simulink model "hdlcodercpu_eml"  (R2026a)
settings: Solver=FixedStepDiscrete  StopTime=20000
libraries: hdlsllib x1
Description:
  | 8-bit RISC Processor using MATLAB(R) Function Blocks
  | This model shows how to use Simulink(R) HDL Coder(TM) to check,
  | generate and verify HDL for an 8-bit CPU implemented using the
  | MATLAB Function Block.
settings Model: ExtModeAutoUpdateStatusClock=off  Creator=The MathWorks, Inc.  LastModifiedBy=The MathWorks, Inc.
settings SolverCC: InsertRTBMode=Auto
settings OptimizationCC: ConditionallyExecuteInputs=off  InitFltsAndDblsToZero=on  EfficientMapNaN2IntZero=off
settings DebuggingCC: AlgebraicLoopMsg=error  UnderspecifiedInitializationDetection=Classic  SingleTaskRateTransMsg=error
settings HardwareCC: ProdHWDeviceType=ASIC/FPGA->ASIC/FPGA  ProdEqTarget=off
settings GRTTargetCC: TargetFcnLib=ansi_tfl_tmw.mat  CombineOutputUpdateFcns=off  GRTInterface=on
settings ConfigComp: DVMaxProcessTime=600.0  DVAutomaticStubbing=off  DVParameterConfiguration=UseParameterConfigFile  DVParameters=on  DVModelCoverageObjectives=MCDC  DVMaxTestCaseSteps=500.0  DVTestSuiteOptimization=Auto  DVAbsoluteTolerance=1.0e-5  DVDefectChecker=off  DVDetectActiveLogic=on  DVMaxViolationSteps=20.0  DVSaveHarnessModel=on  DVModelReferenceHarness=on  DVHarnessSource=Signal Editor  DVSaveReport=on  DVActiveTab=0.0

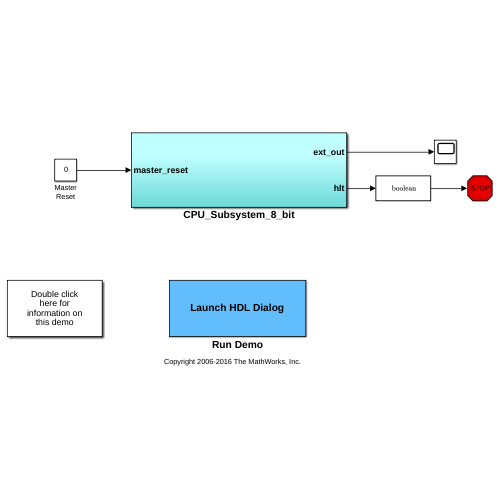
[thumbnail: Simulink's stored preview of the top-level diagram]
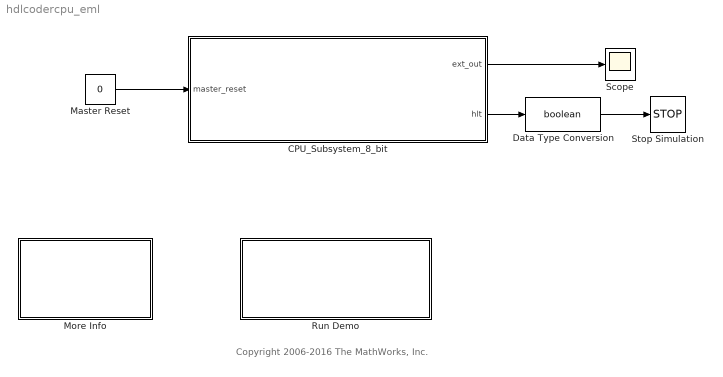
== system hdlcodercpu_eml ==
  note: Copyright 2006-2016 The MathWorks, Inc.
  CPU_Subsystem_8_bit : Subsystem
  Data Type Conversion : DataTypeConversion  OutDataTypeStr=boolean  SaturateOnIntegerOverflow=off  RndMeth=Floor
  Master Reset : Constant  Value=0  OutDataTypeStr=boolean  SampleTime=1
  More Info : Subsystem
      mask Display: disp('Double click\nhere for\ninformation on\nthis demo')
  Run Demo : Subsystem
      settings: OpenFcn=hdldialog(bdroot)
      mask Display: disp('Launch HDL Dialog')
  Scope : Scope
      settings: TimeSpan=100  ActiveDisplayYMinimum=0  ActiveDisplayYMaximum=7  DataLoggingMaxPoints=8500
  Stop Simulation : Stop
  wires:
  CPU_Subsystem_8_bit/1(ext_out) -> Scope/1
  CPU_Subsystem_8_bit/2(hlt) -> Data Type Conversion/1
  Data Type Conversion/1 -> Stop Simulation/1
  Master Reset/1 -> CPU_Subsystem_8_bit/1(master_reset)

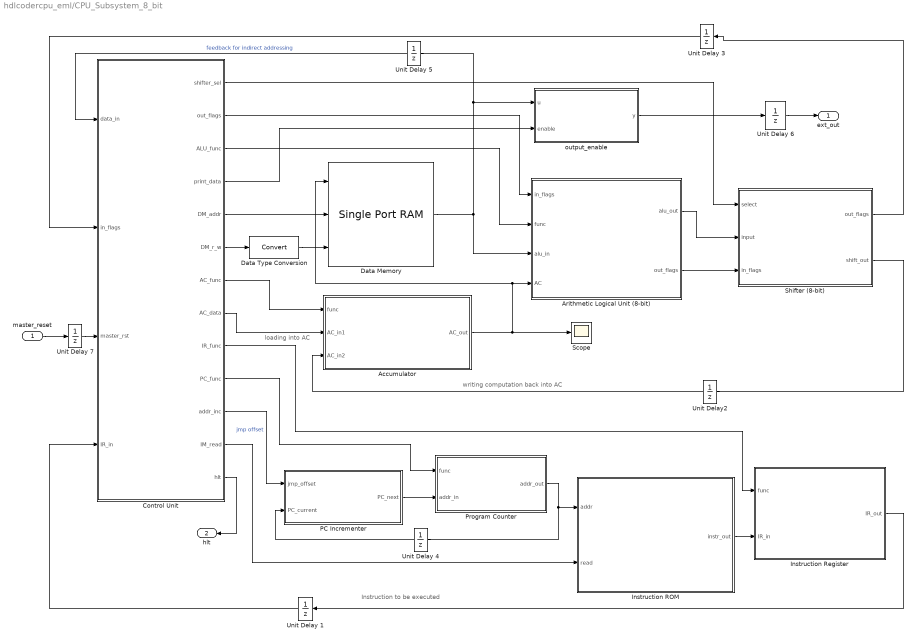
== system hdlcodercpu_eml/CPU_Subsystem_8_bit ==
  note: loading into AC
  note: writing computation back into AC
  note: Instruction to be executed
  master_reset : Inport
  Accumulator : MATLAB Function  TreatAsAtomicUnit=on
  Arithmetic Logical Unit (8-bit) : MATLAB Function  TreatAsAtomicUnit=on
  Control Unit : MATLAB Function  TreatAsAtomicUnit=on
  Data Memory : hdlsllib/HDL RAMs/Single Port RAM  ram_size=8  dout_type=New data
  Data Type Conversion : DataTypeConversion  SaturateOnIntegerOverflow=off  RndMeth=Floor
  Instruction ROM : MATLAB Function  TreatAsAtomicUnit=on
  Instruction Register : MATLAB Function  TreatAsAtomicUnit=on
  PC Incrementer : MATLAB Function  TreatAsAtomicUnit=on
  Program Counter : MATLAB Function  TreatAsAtomicUnit=on
  Scope : Scope
  Shifter (8-bit) : MATLAB Function  TreatAsAtomicUnit=on
  Unit Delay {1,3..7} (6 alike) : UnitDelay
  Unit Delay2 : UnitDelay
  output_enable : MATLAB Function  TreatAsAtomicUnit=on
  ext_out : Outport
  hlt : Outport  Port=2
  wires:
  Arithmetic Logical Unit (8-bit)/1(alu_out) -> Shifter (8-bit)/2(input)
  Arithmetic Logical Unit (8-bit)/2(out_flags) -> Shifter (8-bit)/3(in_flags)
  Accumulator/1(AC_out) -> Arithmetic Logical Unit (8-bit)/4(AC), Data Memory/1, Scope/1
  Data Memory/1 -> Arithmetic Logical Unit (8-bit)/3(alu_in), output_enable/1(u), Unit Delay 5/1
  Program Counter/1(addr_out) -> Instruction ROM/1(addr), Unit Delay 4/1
  PC Incrementer/1(PC_next) -> Program Counter/2(addr_in)
  Instruction ROM/1(instr_out) -> Instruction Register/2(IR_in)
  Control Unit/3(ALU_func) -> Arithmetic Logical Unit (8-bit)/2(func)
  Control Unit/1(shifter_sel) -> Shifter (8-bit)/1(select)
  Control Unit/2(out_flags) -> Arithmetic Logical Unit (8-bit)/1(in_flags)
  Control Unit/6(DM_r_w) -> Data Type Conversion/1
  Control Unit/7(AC_func) -> Accumulator/1(func)
  Control Unit/9(IR_func) -> Instruction Register/1(func)
  Control Unit/10(PC_func) -> Program Counter/1(func)
  Control Unit/11(addr_inc) -> PC Incrementer/1(jmp_offset)  "jmp offset"
  Control Unit/12(IM_read) -> Instruction ROM/2(read)
  Instruction Register/1(IR_out) -> Unit Delay 1/1
  Shifter (8-bit)/2(shift_out) -> Unit Delay2/1
  Unit Delay2/1 -> Accumulator/3(AC_in2)
  Unit Delay 4/1 -> PC Incrementer/2(PC_current)
  Control Unit/8(AC_data) -> Accumulator/2(AC_in1)
  master_reset/1 -> Unit Delay 7/1
  Control Unit/4(print_data) -> output_enable/2(enable)
  Control Unit/13(hlt) -> hlt/1
  Unit Delay 5/1 -> Control Unit/1(data_in)  "feedback for indirect addressing"
  output_enable/1(y) -> Unit Delay 6/1
  Data Type Conversion/1 -> Data Memory/3
  Control Unit/5(DM_addr) -> Data Memory/2
  Unit Delay 6/1 -> ext_out/1
  Unit Delay 7/1 -> Control Unit/3(master_rst)
  Unit Delay 3/1 -> Control Unit/2(in_flags)
  Unit Delay 1/1 -> Control Unit/4(IR_in)
  Shifter (8-bit)/1(out_flags) -> Unit Delay 3/1

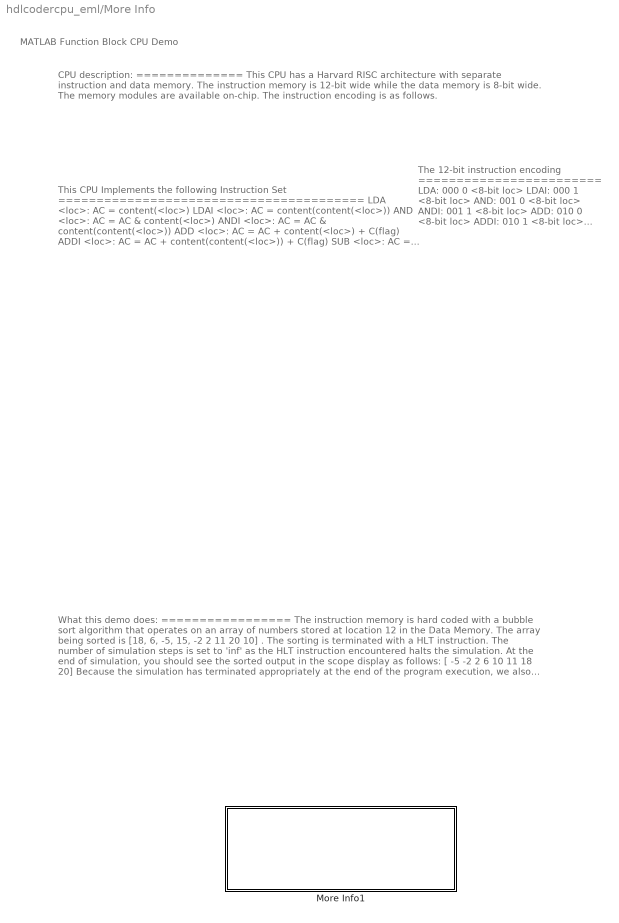
== system hdlcodercpu_eml/More Info ==
  note: MATLAB Function Block CPU Demo
  note: This CPU Implements the following Instruction Set
      | ========================================
      |
      | LDA <loc>: AC = content(<loc>)
      | LDAI <loc>: AC = content(content(<loc>))
      | AND <loc>: AC = AC & content(<loc>)
      | ANDI <loc>: AC = AC & content(content(<loc>))
      | ADD <loc>: AC = AC + content(<loc>) + C(flag)
      | ADDI <loc>: AC = AC + content(content(<loc>)) + C(flag)
      | SUB <loc>: AC = AC - content(<loc>) - C(flag)
      | SUBI <loc>: AC = AC - content(content(<loc>)) - C(flag)
      | JMP <loc>: Jump to <PC + <loc>>
      | LI <const>: AC = <const>
      | STA <loc>: content(<loc>) = AC
      | STAI <loc>: content(content(<loc>)) = AC
      | BRA_C <loc>: Jump to <PC + <loc>> if (C(flag) == 1)
      | BRA_N <loc>: Jump to <PC + <loc>> if (N(flag) == 1)
      | BRA_V <loc>: Jump to <PC + <loc>> if (V(flag) == 1)
      | BRA_Z <loc>: Jump to <PC + <loc>> if (Z(flag) == 1)
      | HLT: Halt (simulation)
      | CLA: AC = 0
      | CMA: Complement AC
      | CMC: Complement C(flag)
      | ASL: AC = AC << 1
      | ASR: AC = AC >> 1
      | PRINT: Display value from the memory-mapped location 255
      | CLC: C(flag) = 0
  note: The 12-bit instruction encoding
      | ========================
      |
      | LDA:     000 0 <8-bit loc>
      | LDAI:    000 1 <8-bit loc>
      | AND:     001 0 <8-bit loc>
      | ANDI:    001 1 <8-bit loc>
      | ADD:     010 0 <8-bit loc>
      | ADDI:    010 1 <8-bit loc>
      | SUB:     011 0 <8-bit loc>
      | SUBI:    011 1 <8-bit loc>
      | JMP:     1000 <8-bit loc>
      | LI:         1001 <8-bit const>
      | STA:     101 0 <8-bit loc>
      | STAI:    101 1 <8-bit loc>
      | BRA_C: 1100 <8-bit loc>
      | BRA_N: 1101 <8-bit loc>
      | BRA_C: 1110 <8-bit loc>
      | BRA_C: 1111 <8-bit loc>
      | HLT:     111 0 0100 0 000
      | CLA:      111 0 0100 1 000
      | CMA:     111 0 0101 0 000
      | CMC:     111 0 0101 1 000
      | ASL:      111 0 0110 0 000
      | ASR:      111 0 0110 1 000
      | PRINT:  111 0 0111 0 000
      | CLC:      111 0 0111 1 000
  note: CPU description:
      | ==============
      |
      | This CPU has a Harvard RISC architecture with separate instruction and data memory.
      | The instruction memory is 12-bit wide while the data memory is 8-bit wide.
      | The memory modules are available on-chip. The instruction encoding is as follows.
  note: What this demo does:
      | =================
      | The instruction memory is hard coded with a bubble sort algorithm that operates on an array
      | of numbers stored at location 12 in the Data Memory. The array being sorted is
      | [18, 6, -5, 15, -2 2 11 20 10] . The sorting is terminated with a HLT instruction.
      |
      | The number of simulation steps is set to 'inf' as the HLT instruction encountered halts the
      | simulation. At the end of simulation, you should see the sorted output in the scope display
      | as follows: [ -5 -2 2 6 10 11 18 20]
      |
      | Because the simulation has terminated appropriately at the end of the program execution,
      | we also get the number of time steps needed to execute the program.
  More Info1 : Subsystem
      mask Display: disp('Details of the Instruction memory\nthat contains a bubble sort algorithm')

== system hdlcodercpu_eml/Run Demo ==

== system hdlcodercpu_eml/More Info/More Info1 ==
  note: Bubble Sort
      | =========
      |
      | % Array Size
      |   LI 10     %  n = 10
      |   STA 0     %  n in loc 0
      |
      | % Array Pointer
      |   LI 12      %  loc 12 = starting location of a[]
      |   STA 1     %  loc 1 stores i which points to a[]
      |
      | % Array Entries begin in loc 12
      |   LI 18
      |   STA 12   % entry 1
      |   LI 6
      |   STA 13   % entry 2
      |   LI 19
      |   STA 14   % entry 3
      |   LI -5
      |   STA 15   % entry 4
      |   LI 15
      |   STA 16   % entry 5
      |   LI -2
      |   STA 17   % entry 6
      |   LI 2
      |   STA 18   % entry 7
      |   LI 11
      |   STA 19   % entry 8
      |   LI 20
      |   STA 20   % entry 9
      |   LI 10
      |   STA 21   % entry 10
      | L1:
      |   LI 1
      |   STA 2     %  loc 2 keeps track of count
      |   LI 1
      |   STA 3     %  loc 3 contains a predicate to flag the end of sorting
      | L2:
      | % accessing a[i-1]
      |   LI 1
      |   STA 4
      |   LDA 2
      |   CLC
      |   SUB 4    % i-1
      |   CLC
      |   ADD 1
      |   STA 5   % storing i-1 in loc 5
      |   LDAI 5   % a[i-1]
      |   STA 6    % temporarily storing a[i-1] in loc 6
      | % accessing a[i]
      |   LDA 2
      |   CLC
      |   ADD 1
      |   STA 7   % storing i in loc 7
      |   LDAI 7   % a[i]
      |   CLC
      |   SUB 6  % a[i] - a[i-1]
      |   BRA_N L5
      |   % a[i] >= a[i-1]
      |   JMP L6
  note: Bubble Sort     (continued)
      | =========
      |  L5:
      |    % a[i-1] > a[i]
      |  %  reset the flag indicating further sorting passes are reqd
      |    LI 0
      |    STA 3
      |  % Swapping a[i] and a[i-1]
      |    LDAI 7   % a[i]
      |    STAI 5   % a[i-1] = a[i]
      |    LDA 6   % temp
      |    STAI 7   % a[i] = temp
      |  L6:
      |    LI 1
      |    CLC
      |    ADD 2
      |    STA 2     %  count = count + 1
      |    LDA 0
      |    CLC
      |    SUB 2    %  AC = n - count
      |    BRA_Z L3    %  Break out of loop if count == n
      |    JMP L2
      |  L3:
      |    LI 1
      |    STA 4
      |    LDA 3
      |    CLC
      |    SUB 4
      |    BRA_Z L4    %  if flag == 1 indicating sorting over, break out
      |    JMP L1
      |  L4:
      |    LI 0
      |    STA 2     %  loc 2 keeps track of count
      |  % Printing the array
      |  L7:
      |    LDAI 1   % load a[i]
      |    STA 255
      |    PRINT     %  printing a[i]
      |    LI 1
      |    CLC
      |    ADD 1
      |    STA 1     %  i = i + 1
      |    LI 1
      |    CLC
      |    ADD 2
      |    STA 2     %  count = count + 1
      |    LDA 0
      |    CLC
      |    SUB 2    %  AC = n - count
      |    BRA_Z L8    %  Break out of loop if count == n
      |    JMP L7    %  Looping around
      |  L8:
      |    HLT
  note: The following program is hardcoded in
      | hdlcodercpu_eml/CPU Subsystem (8-bit)/Instruction ROM

== matlab function hdlcodercpu_eml/CPU_Subsystem_8_bit/PC Incrementer ==
  settings: updateMethod=DISCRETE  sampleTime=1
  settings: fimath=|
      | fimath(...
      | 'RoundMode', 'floor',...
      | 'OverflowMode', 'wrap',...
      | 'ProductMode', 'FullPrecision', 'ProductWordLength', 32,...
      | 'SumMode', 'FullPrecision', 'SumWordLength', 32,...
      | 'CastBeforeSum', true)
  data: jmp_offset input fixdt(1,8,0); PC_current input fixdt(0,8,0); PC_next output
function PC_next  = PC_Inc(jmp_offset, PC_current)
% PC incrementer increments the PC with jmp_offset

% HDL specific fimath
hdl_fm = fimath(...
'RoundMode', 'floor',...
'OverflowMode', 'wrap',...
'ProductMode', 'FullPrecision', 'ProductWordLength', 32,...
'SumMode', 'FullPrecision', 'SumWordLength', 32,...
'CastBeforeSum', true);

PC_next = fi(jmp_offset + PC_current, 0, 8, 0, hdl_fm);

== matlab function hdlcodercpu_eml/CPU_Subsystem_8_bit/output_enable ==
  data: u input fixdt(1,8,0); y output; enable input
function y = output_enable(u, enable)
% to the pin-out

% HDL specific fimath
hdl_fm = fimath(...
'RoundMode', 'floor',...
'OverflowMode', 'wrap',...
'ProductMode', 'FullPrecision', 'ProductWordLength', 32,...
'SumMode', 'FullPrecision', 'SumWordLength', 32,...
'CastBeforeSum', true);

y = fi(0, 1, 8, 0, hdl_fm);

if(enable)
    y = fi(u, 1, 8, 0, hdl_fm);
end

== matlab function hdlcodercpu_eml/CPU_Subsystem_8_bit/Control Unit ==
  settings: updateMethod=DISCRETE  sampleTime=1
  settings: fimath=|
      | fimath(...
      | 'RoundMode', 'floor',...
      | 'OverflowMode', 'wrap',...
      | 'ProductMode', 'FullPrecision', 'ProductWordLength', 32,...
      | 'SumMode', 'FullPrecision', 'SumWordLength', 32,...
      | 'CastBeforeSum', true)
  data: data_in input fixdt(1,8,0); in_flags input fixdt(0,4,0); master_rst input; shifter_sel output; out_flags output; ALU_func output; print_data output; IR_in input fixdt(0,12,0); DM_addr output; DM_r_w output; AC_func output; AC_data output; IR_func output; PC_func output; addr_inc output; IM_read output; hlt output
function [shifter_sel, out_flags, ALU_func, ...
    print_data, DM_addr, DM_r_w, AC_func, AC_data, IR_func, ...
    PC_func, addr_inc, IM_read, hlt] = Controller(data_in, in_flags, master_rst, IR_in)
% CPU Controller
%
% The CPU Instruction Set:
% ------------------------
% 
% LDA <loc>: AC = content(<loc>)
% LDAI <loc>: AC = content(content(<loc>))
% AND <loc>: AC = AC & content(<loc>)
% ANDI <loc>: AC = AC & content(content(<loc>))
% ADD <loc>: AC = AC + content(<loc>) + C(flag) 
% ADDI <loc>: AC = AC + content(content(<loc>)) + C(flag)
% SUB <loc>: AC = AC - content(<loc>) - C(flag) 
% SUBI <loc>: AC = AC - content(content(<loc>)) - C(flag)
% JMP <loc>: Jump to <PC + <loc>>
% LI <const>: AC = <const>
% STA <loc>: content(<loc>) = AC
% STAI <loc>: content(content(<loc>)) = AC
% BRA_C <loc>: Jump to <PC + <loc>> if (C(flag) == 1)
% BRA_N <loc>: Jump to <PC + <loc>> if (N(flag) == 1)
% BRA_V <loc>: Jump to <PC + <loc>> if (V(flag) == 1)
% BRA_Z <loc>: Jump to <PC + <loc>> if (Z(flag) == 1)
% NOP: Do nothing
% CLA: AC = 0
% CMA: Complement AC
% CMC: Complement C(flag)
% ASL: AC = AC << 1
% ASR: AC = AC >> 1
% PRINT: Display value from the memory-mapped location 255
% CLC: C(flag) = 0
%
% 12-bit Instruction Encoding:
% ---------------------------
%
% 	LDA:   000 0 <8-bit loc>
% 	LDAI:  000 1 <8-bit loc>
% 	AND:   001 0 <8-bit loc>
% 	ANDI:  001 1 <8-bit loc>
% 	ADD:   010 0 <8-bit loc>
% 	ADDI:  010 1 <8-bit loc>
% 	SUB:   011 0 <8-bit loc>
% 	SUBI:  011 1 <8-bit loc>
% 	JMP:   1000 <8-bit loc>
% 	LI:    1001 <8-bit const>
% 	STA:   101 0 <8-bit loc>
% 	STAI:  101 1 <8-bit loc>
% 	BRA_C: 1100 <8-bit loc>
% 	BRA_N: 1101 <8-bit loc>
% 	BRA_C: 1110 <8-bit loc>
% 	BRA_C: 1111 <8-bit loc>
% 	HLT:   111 0 0100 0 000 
% 	CLA:   111 0 0100 1 000
% 	CMA:   111 0 0101 0 000
% 	CMC:   111 0 0101 1 000
% 	ASL:   111 0 0110 0 000
% 	ASR:   111 0 0110 1 000
% 	PRINT: 111 0 0111 0 000
% 	CLC:   111 0 0111 1 000  

% HDL specific fimath
hdl_fm = fimath(...
'RoundMode', 'floor',...
'OverflowMode', 'wrap',...
'ProductMode', 'FullPrecision', 'ProductWordLength', 32,...
'SumMode', 'FullPrecision', 'SumWordLength', 32,...
'CastBeforeSum', true);


persistent CPU_state;
if(isempty(CPU_state))
    CPU_state = uint8(0);
end

persistent previous_CPU_state;
if(isempty(previous_CPU_state))
    previous_CPU_state = uint8(0);
end

if(master_rst)
    CPU_state = uint8(0);
end

shifter_sel = fi(0, 0, 2, 0, hdl_fm);
ALU_func = fi(0, 0, 3, 0, hdl_fm);
out_flags = in_flags;
AC_func = fi(4, 0, 3, 0, hdl_fm);  % NOP
AC_data = fi(0, 1, 8, 0, hdl_fm);
IR_func = fi(3, 0, 2, 0, hdl_fm);  % NOP
PC_func = fi(3, 0, 2, 0, hdl_fm);  % NOP
IM_read = fi(0, 0, 1, 0, hdl_fm);
DM_addr = fi(0, 0, 8, 0, hdl_fm); % uint8(0)
DM_r_w = fi(0, 0, 1, 0, hdl_fm);
addr_inc = fi(0, 1, 8, 0, hdl_fm);
print_data = false;
hlt = uint8(0);

% Instruction: <12..1>
% major_opcode: <12..10>
% indirect_addressing: <9>
% minor_opcode: <9..4>
% address bits: <8..1>

persistent major_opcode; 
persistent minor_opcode; 
persistent address_data;
persistent indirect_address;

if(isempty(major_opcode))
    major_opcode = fi(0, 0, 8, 0, hdl_fm);
    minor_opcode = fi(0, 0, 8, 0, hdl_fm);
    address_data = fi(0, 0, 8, 0, hdl_fm);
    indirect_address = fi(0, 0, 8, 0, hdl_fm);
end

switch(CPU_state)
    %%%%%%%%%%%%%%%%%%%%%%%%%%%%%%%%%%%%%%
    %  RESETTING OUTPUTS
    %%%%%%%%%%%%%%%%%%%%%%%%%%%%%%%%%%%%%%
    case 0
        PC_func = fi(0, 0, 2, 0, hdl_fm);   
        AC_func = fi(0, 0, 3, 0, hdl_fm);   
        IR_func = fi(0, 0, 2, 0, hdl_fm);   
        previous_CPU_state = CPU_state;
        CPU_state = uint8(1);
        
    %%%%%%%%%%%%%%%%%%%%%%%%%%%%%%%%%%%%%%
    %  FETCH
    %%%%%%%%%%%%%%%%%%%%%%%%%%%%%%%%%%%%%%
    case 1  
        % Read from IM
        IM_read = fi(1, 0, 1, 0, hdl_fm);  
        % Increment PC
        PC_func = fi(2, 0, 2, 0, hdl_fm);  
        % store into IR
        IR_func = fi(1, 0, 2, 0, hdl_fm);  
        
        CPU_state = uint8(2);
        
    case 2 
        % Read from IR
        IR_func = fi(2, 0, 2, 0, hdl_fm);  
        % Accommodating for the 'unit delay' from IR_out to IR_in
        
        CPU_state = uint8(3);  
        
    case 3
        % IR_in <12..10>
        major_opcode = fi(bitsrl(IR_in, 9), 0, 8, 0, hdl_fm);
        mask = fi(63, 0, 12, 0, hdl_fm);
        % IR_in <9..4>
        minor_opcode = fi(bitand(bitsrl(IR_in, 3), mask), 0, 8, 0, hdl_fm);
        mask = fi(255, 0, 12, 0, hdl_fm);
        % IR_in <8..1>
        address_data = fi(bitand(IR_in, mask), 0, 8, 0, hdl_fm);
        
        % Go to the decode stage
        CPU_state = uint8(4);  
        
    %%%%%%%%%%%%%%%%%%%%%%%%%%%%%%%%%%%%%%
    %  DECODE AND EXECUTE
    %%%%%%%%%%%%%%%%%%%%%%%%%%%%%%%%%%%%%%
    case 4  
        previous_CPU_state = CPU_state;
        switch(uint8(major_opcode))
            case 0  
                % LDA
                % minor_opcode contains the address (assuming direct addressing)
                DM_addr = address_data; 
                % Read the data memory
                DM_r_w = fi(0, 0, 1, 0, hdl_fm); 
                % Simply pass the value read from memory
                CPU_state = uint8(13);
                
            case 1  
                % AND           
                DM_addr = address_data;
                % Reading the data memory for address or data
                DM_r_w = fi(0, 0, 1, 0, hdl_fm);
                
                CPU_state = uint8(15);
                
            case 2  
                % ADD
                DM_addr = address_data;
                % Reading the data memory for address or data
                DM_r_w = fi(0, 0, 1, 0, hdl_fm);
                
                CPU_state = uint8(17);
                
            case 3  
                % SUB
                DM_addr = address_data;
                % Reading the data memory for address or data
                DM_r_w = fi(0, 0, 1, 0, hdl_fm);
                
                CPU_state = uint8(19);

            case 4  
                minor_opcode_bit6 = bitget(minor_opcode, 6);
                switch(uint8(minor_opcode_bit6))
                    case 0 
                        % JMP
                        temp_address_data = fi(address_data, 1, 7, 0, hdl_fm);
                        addr_inc = fi(temp_address_data-1, 1, 8, 0, hdl_fm);
                        PC_func = fi(1, 0, 2, 0, hdl_fm); 
                        
                    case 1
                        % LI
                        AC_data = fi(address_data, 1, 8, 0, hdl_fm);
                        AC_func = fi(1, 0, 3, 0, hdl_fm);
                end
                % Go back to the fetch stage again
                CPU_state = uint8(1);  
                
            case 5  
                % STA
                % minor_opcode contains the address (assuming direct addressing)
                DM_addr = address_data; 
                indirect_bit = bitget(minor_opcode, 6);
                if(logical(indirect_bit))
                    % indirect addressing
                    % Read the address from the data memory
                    DM_r_w = fi(0, 0, 1, 0, hdl_fm); 
                    CPU_state = uint8(21);
                else
                    % Write into the data memory
                    DM_r_w = fi(1, 0, 1, 0, hdl_fm);
                    % Go back to the fetch stage again
                    CPU_state = uint8(25);  % going to 'otherwise'
                end
                
            case 6
                minor_opcode_bit6 = bitget(minor_opcode, 6);
                switch(uint8(minor_opcode_bit6))
                    % special branches:
                    case 0 
                        % BRA_C
                        c = bitget(in_flags, 4);
                        if(logical(c))
                            temp_address_data = fi(address_data, 1, 7, 0, hdl_fm);
                            addr_inc = fi(temp_address_data-1, 1, 8, 0, hdl_fm);
                            PC_func = fi(1, 0, 2, 0, hdl_fm);
                        end
                        
                    case 1
                        % BRA_N
                        n = bitget(in_flags, 3);
                        if(logical(n))
                            temp_address_data = fi(address_data, 1, 7, 0, hdl_fm);
                            addr_inc = fi(temp_address_data-1, 1, 8, 0, hdl_fm);
                            PC_func = fi(1, 0, 2, 0, hdl_fm);
                        end
                end
                % Go back to the fetch stage again
                CPU_state = uint8(15);
                
            case 7  
                 % by default, go back to the fetch stage again
                CPU_state = uint8(1);
                minor_opcode_bit4 = bitget(minor_opcode, 4);
                if(logical(minor_opcode_bit4) == 0)
                    % Further cases of special branches:
                    minor_opcode_bit6 = bitget(minor_opcode, 6);
                    switch(uint8(minor_opcode_bit6))
                        case 0 
                            % BRA_V
                            v = bitget(in_flags, 2);
                            if(logical(v))
                                temp_address_data = fi(address_data, 1, 7, 0, hdl_fm);
                                addr_inc = fi(temp_address_data-1, 1, 8, 0, hdl_fm);
                                PC_func = fi(1, 0, 2, 0, hdl_fm);
                            end
                         
                        case 1 
                            % BRA_Z
                            z = bitget(in_flags, 1);
                            if(logical(z))
                                temp_address_data = fi(address_data, 1, 7, 0, hdl_fm);
                                addr_inc = fi(temp_address_data-1, 1, 8, 0, hdl_fm);
                                PC_func = fi(1, 0, 2, 0, hdl_fm);
                            end
                    end
                end
                % Instructions having no operands
                switch(uint8(minor_opcode))
                    case 8
                        % HLT
                        % Stop the simulation
                        hlt = uint8(1);
                        CPU_state = uint8(22);
                    case 9 
                        % CLA
                        AC_func = fi(0, 0, 3, 0, hdl_fm);
                        
                    case 10 
                        % CMA
                        ALU_func = fi(4, 0, 3, 0, hdl_fm); 
                        shifter_sel = fi(3, 0, 2, 0, hdl_fm);
                        CPU_state = uint8(6);
                        
                    case 11 
                        % CMC
                        ALU_func = fi(5, 0, 3, 0, hdl_fm); 
                        shifter_sel = fi(3, 0, 2, 0, hdl_fm);
                        
                    case 12 
                        % ASL
                        shifter_sel = fi(1, 0, 2, 0, hdl_fm);
                        CPU_state = uint8(6);
                        
                    case 13 
                        % ASR
                        shifter_sel = fi(2, 0, 2, 0, hdl_fm);
                        CPU_state = uint8(6);
                        
                    case 14 
                        % PRINT   
                        DM_addr = fi(255, 0, 8, 0, hdl_fm);
                        % Read the data memory
                        DM_r_w = fi(0, 0, 1, 0, hdl_fm);
                        
                        CPU_state = uint8(12);

                    case 15 
                        % CLC
                        ALU_func = fi(7, 0, 3, 0, hdl_fm); 
                        shifter_sel = fi(3, 0, 2, 0, hdl_fm);
                        
                    otherwise
                        % by default, go back to the fetch stage again
                        CPU_state = uint8(1);
  
                % Minor Opcode cases end here        
                end
        % Major Opcode cases end here
        end
    
    % introducing delay
    case 6
        % accounting for the delay from shift_out to AC_in2
        AC_func = fi(2, 0, 3, 0, hdl_fm);
        previous_CPU_state = CPU_state;
        % Go back to the fetch stage again
        CPU_state = uint8(1);  
        
    % Operations with indirect addressing
    case 7
        % LDA Indirect
        % data_in is the address read from the data memory
        DM_addr = indirect_address; 
        % Read the data memory
        DM_r_w = fi(0, 0, 1, 0, hdl_fm); 
        
        previous_CPU_state = CPU_state;
        CPU_state = uint8(13);
        
    case 8
        % AND Indirect
        % data_in is the address read from the data memory
        DM_addr = indirect_address;
        % Read the data memory
        DM_r_w = fi(0, 0, 1, 0, hdl_fm);

        previous_CPU_state = CPU_state;
        CPU_state = uint8(15);
    
    case 9
        % ADD Indirect
        % data_in is the address read from the data memory
        DM_addr = indirect_address;
        % Read the data memory
        DM_r_w = fi(0, 0, 1, 0, hdl_fm);
        
        previous_CPU_state = CPU_state;
        CPU_state = uint8(17);
        
    case 10
        % SUB Indirect
        % data_in is the address read from the data memory
        DM_addr = indirect_address;
        % Read the data memory
        DM_r_w = fi(0, 0, 1, 0, hdl_fm);
        
        previous_CPU_state = CPU_state;
        CPU_state = uint8(19);
        
    case 11
        % STA Indirect
        % data_in is the address read from the data memory
        DM_addr = fi(data_in, 0, 8, 0, hdl_fm);
        % Write the data memory
        DM_r_w = fi(1, 0, 1, 0, hdl_fm);
        previous_CPU_state = CPU_state;
        CPU_state = uint8(1);
        
    case 12
        % PRINT
        print_data = true;
        previous_CPU_state = CPU_state;
        CPU_state = uint8(1);
        
    case 13
        % LDA (contd.)
        % Simply pass the value read from memory
        ALU_func = fi(6, 0, 3, 0, hdl_fm);
        shifter_sel = fi(3, 0, 2, 0, hdl_fm);

        if(previous_CPU_state == uint8(4))
            previous_CPU_state = CPU_state;
            CPU_state = uint8(14);
        else
            previous_CPU_state = CPU_state;
            CPU_state = uint8(6);
        end
        
    case 14
        indirect_bit = bitget(minor_opcode, 6);
        % accounting for the delay from shift_out to AC_in2
        AC_func = fi(2, 0, 3, 0, hdl_fm);
        
        previous_CPU_state = CPU_state;
        if(logical(indirect_bit))
            % indirect addressing
            indirect_address = fi(data_in, 0, 8, 0, hdl_fm);
            CPU_state = uint8(7);
        else
            CPU_state = uint8(25);
        end

    case 15

        % AND (contd.)
        ALU_func = fi(1, 0, 3, 0, hdl_fm);
        shifter_sel = fi(3, 0, 2, 0, hdl_fm);

        if(previous_CPU_state == uint8(4))
            previous_CPU_state = CPU_state;
            CPU_state = uint8(16);
        else
            previous_CPU_state = CPU_state;
            CPU_state = uint8(6);
        end

    case 16
        indirect_bit = bitget(minor_opcode, 6);
        % accounting for the delay from shift_out to AC_in2
        AC_func = fi(2, 0, 3, 0, hdl_fm);
        
        previous_CPU_state = CPU_state;
        if(logical(indirect_bit))
            % indirect addressing
            indirect_address = fi(data_in, 0, 8, 0, hdl_fm);
            CPU_state = uint8(8);
        else
            CPU_state = uint8(25);
        end
        
    case 17
        % ADD (contd.)
        ALU_func = fi(2, 0, 3, 0, hdl_fm);
        shifter_sel = fi(3, 0, 2, 0, hdl_fm);

        if(previous_CPU_state == uint8(4))
            previous_CPU_state = CPU_state;
            CPU_state = uint8(18);
        else
            previous_CPU_state = CPU_state;
            CPU_state = uint8(6);
        end

    case 18
        indirect_bit = bitget(minor_opcode, 6);
        % accounting for the delay from shift_out to AC_in2
        AC_func = fi(2, 0, 3, 0, hdl_fm);
        
        previous_CPU_state = CPU_state;
        if(logical(indirect_bit))
            % indirect addressing
            indirect_address = fi(data_in, 0, 8, 0, hdl_fm);
            CPU_state = uint8(9);
        else
            CPU_state = uint8(25);
        end
        
    case 19
        % SUB (contd.)
        ALU_func = fi(3, 0, 3, 0, hdl_fm);
        shifter_sel = fi(3, 0, 2, 0, hdl_fm);

        if(previous_CPU_state == uint8(4))
            previous_CPU_state = CPU_state;
            CPU_state = uint8(20);
        else
            previous_CPU_state = CPU_state;
            CPU_state = uint8(6);
        end

    case 20
        indirect_bit = bitget(minor_opcode, 6);
        % accounting for the delay from shift_out to AC_in2
        AC_func = fi(2, 0, 3, 0, hdl_fm);
        
        previous_CPU_state = CPU_state;
        if(logical(indirect_bit))
            % indirect addressing
            indirect_address = fi(data_in, 0, 8, 0, hdl_fm);
            CPU_state = uint8(10);
        else

            CPU_state = uint8(25);
        end
        
    case 21
        % STA indirect
        CPU_state = uint8(11);
        
    case 22
        % lock state
        hlt = uint8(1);
        CPU_state = uint8(22);

    otherwise
        previous_CPU_state = CPU_state;
        % by default, go back to the fetch stage again
        CPU_state = uint8(1);
                
% switch(CPU_state) end here
end

== matlab function hdlcodercpu_eml/CPU_Subsystem_8_bit/Accumulator ==
  settings: updateMethod=DISCRETE  sampleTime=1
  settings: fimath=|
      | fimath(...
      | 'RoundMode', 'floor',...
      | 'OverflowMode', 'wrap',...
      | 'ProductMode', 'FullPrecision', 'ProductWordLength', 32,...
      | 'SumMode', 'FullPrecision', 'SumWordLength', 32,...
      | 'CastBeforeSum', true)
  data: func input; AC_out output fixdt(1,8,0); AC_in1 input fixdt(1,8,0); AC_in2 input fixdt(1,8,0)

%% Accumulator with the following func:
% func == 0 => reset
% func == 1 => store into AC from port 1
% func == 2 => store into AC from port 2
% func == 3 => read from AC;
% otherwise, preserve old value and return 0
function AC_out = Accumulator(func, AC_in1, AC_in2)

% HDL specific fimath
hdl_fm = fimath(...
'RoundMode', 'floor',...
'OverflowMode', 'wrap',...
'ProductMode', 'FullPrecision', 'ProductWordLength', 32,...
'SumMode', 'FullPrecision', 'SumWordLength', 32,...
'CastBeforeSum', true);


persistent AC_value;
if(isempty(AC_value))
    AC_value = fi(0, 1, 8, 0, hdl_fm);
end

AC_out = fi(AC_value, 1, 8, 0, hdl_fm);
        
switch(uint8(func)) 
    case 0
        % reset
        AC_value = fi(0, 1, 8, 0, hdl_fm); 
    case 1 
        % store into AC
        AC_value = AC_in1;
    case 2
        % store into AC
        AC_value = AC_in2;    
    case 3
        % read the AC value
        AC_out = AC_value;
end

== matlab function hdlcodercpu_eml/CPU_Subsystem_8_bit/Arithmetic Logical Unit (8-bit) ==
  settings: updateMethod=DISCRETE  sampleTime=1
  settings: fimath=|
      | fimath(...
      | 'RoundMode', 'floor',...
      | 'OverflowMode', 'wrap',...
      | 'ProductMode', 'FullPrecision', 'ProductWordLength', 32,...
      | 'SumMode', 'FullPrecision', 'SumWordLength', 32,...
      | 'CastBeforeSum', true)
  data: in_flags input fixdt(0,4,0); func input fixdt(0,3,0); alu_in input fixdt(1,8,0); AC input fixdt(1,8,0); alu_out output fixdt(1,8,0); out_flags output
function [alu_out, out_flags] = ALU(in_flags, func, alu_in, AC)
% This 8-bit ALU supports the following operations:
% AND (Logical AND), ADD, SUB, CMA (Complement AC), CMC (Complement Carry) and CLC (Clear Carry)
% and appropriately sets a 4-bit flag register, which has the following format:
% [C N V Z]

% HDL specific fimath
hdl_fm = fimath(...
'RoundMode', 'floor',...
'OverflowMode', 'wrap',...
'ProductMode', 'FullPrecision', 'ProductWordLength', 32,...
'SumMode', 'FullPrecision', 'SumWordLength', 32,...
'CastBeforeSum', true);

% Get the carry in
carry = bitget(in_flags, 4); 

% Get the overflow in
overflow = bitget(in_flags, 2);

% Simply pass the AC, when there is no designated func
alu_out = fi(AC, 1, 8, 0, hdl_fm);

% 3-bit encoding of ALU ops, which can potentially support upto 8 operations
% Most of the encodings are unused to comply to Parwan supported ops
switch(uint8(func))
    case 0 % NOP
        % simply pass the AC
    case 1 % AND
        % Bitwise AND
        alu_out = bitand(alu_in, AC);
    case 2 % ADD
        % Add with carry and overflow appropriately set
        [alu_out, carry, overflow] = sum_w_carry(AC, alu_in, carry);
    case 3 % SUB
        % Subtract with borrow (set to carry) and overflow appropriately set
        [alu_out, carry, overflow] = sub_w_borrow(AC, alu_in, carry);
    case 4 % CMA
        % Complement AC
        alu_out = fi(bitcmp(AC), 1, 8, 0, hdl_fm);
    case 5 % CMC
        % Complement Carry
        carry = bitcmp(carry);
    case 6 % Get alu_in out
        % Pass the input
        alu_out = fi(alu_in, 1, 8, 0, hdl_fm);
    case 7 % CLC
        % Clear Carry
        carry = fi(0, 0, 1, 0, hdl_fm); 
end

% Negativity  (N)
sign_bit = getmsb(alu_out); 

% Is Zero? (Z)
is_zero = uint8(~all(alu_out));
zero_ufix1 = fi(is_zero, 0, 1, 0, hdl_fm);

% Set the output flag register [C N V Z]
out_flags = bitconcat(bitconcat(bitconcat(carry, sign_bit), overflow), zero_ufix1);

%%%%%%%%%%%%%%%%%%%%%%%%%%%%%%%%%%%%%%%%%%%%%%%%%%%%%%%%%%%%%%%%


%% Full Subtracter with flag register appropriately set 
% diff = u1 - u2 - b_in = u1 + bitcmp(u2) + bitcmp(b_in)
% appropriately set the borrow and the overflow
function [diff, carry, overflow] = sub_w_borrow(u1, u2, b_in)

[diff, carry, overflow] = sum_w_carry(u1, bitcmp(u2), bitcmp(b_in));
%%%%%%%%%%%%%%%%%%%%%%%%%%%%%%%%%%%%%%%%%%%%%%%%%%%%%%%%%%%%%%%%


%% Full Adder with flag register appropriately set
% sum = u1 + u2 + c_in
% appropriately set the carry and the overflow
function [sum, carry, overflow] = sum_w_carry(u1, u2, c_in)

hdl_fm = fimath(...
'RoundMode', 'floor',...
'OverflowMode', 'wrap',...
'ProductMode', 'FullPrecision', 'ProductWordLength', 32,...
'SumMode', 'FullPrecision', 'SumWordLength', 32,...
'CastBeforeSum', true);

% zero-extend u1 by 1 bit for carry detection
temp_u1 = fi(bitconcat(fi(0, 0, 1, 0, hdl_fm), u1), 1, 9, 0, hdl_fm);

% zero-extend u2 by 1 bit for carry detection
temp_u2 = fi(bitconcat(fi(0, 0, 1, 0, hdl_fm), u2), 1, 9, 0, hdl_fm);

% Sum is stored in 9 bits with the msb indicating carry
temp_sum = fi(temp_u1 + temp_u2 + c_in, 1, 9, 0, hdl_fm);

% Carry  (C)
carry = getmsb(temp_sum);

% Stored back in the designated register
sum = fi(temp_sum, 1, 8, 0, hdl_fm);

% Sign bit
sign_bit = getmsb(sum); 

% if the inputs have the same sign and the output generated has a different sign, 
% overflow is generated!
overflow_int = uint8((getmsb(u1) == getmsb(u2)) ...
                     && (sign_bit ~= bitget(u1,8)));
                 
% Overflow (V)
overflow = fi(overflow_int, 0, 1, 0, hdl_fm);

%%%%%%%%%%%%%%%%%%%%%%%%%%%%%%%%%%%%%%%%%%%%%%%%%%%%%%%%%%%%%%%%

== matlab function hdlcodercpu_eml/CPU_Subsystem_8_bit/Instruction ROM ==
  settings: updateMethod=DISCRETE  sampleTime=1
  settings: fimath=|
      | fimath(...
      | 'RoundMode', 'floor',...
      | 'OverflowMode', 'wrap',...
      | 'ProductMode', 'FullPrecision', 'ProductWordLength', 32,...
      | 'SumMode', 'FullPrecision', 'SumWordLength', 32,...
      | 'CastBeforeSum', true)
  data: addr input uint8; read input fixdt(0,1,0); instr_out output
function instr_out = Instr_Memory(addr, read)
%% Instruction Memory

% read == 1 => read from IM

% HDL specific fimath
hdl_fm = fimath(...
'RoundMode', 'floor',...
'OverflowMode', 'wrap',...
'ProductMode', 'FullPrecision', 'ProductWordLength', 32,...
'SumMode', 'FullPrecision', 'SumWordLength', 32,...
'CastBeforeSum', true);


persistent data;
if(isempty(data))
    data = fi(zeros(1, 256), 0, 12, 0, hdl_fm);
end

% ASSEMBLED CODE from sort1.in
data(1) = fi(2314, 0, 12, 0, hdl_fm);    % LI 10
data(2) = fi(2560, 0, 12, 0, hdl_fm);    % STA 0
data(3) = fi(2316, 0, 12, 0, hdl_fm);    % LI 12
data(4) = fi(2561, 0, 12, 0, hdl_fm);    % STA 1
data(5) = fi(2322, 0, 12, 0, hdl_fm);    % LI 18
data(6) = fi(2572, 0, 12, 0, hdl_fm);    % STA 12
data(7) = fi(2310, 0, 12, 0, hdl_fm);    % LI 6
data(8) = fi(2573, 0, 12, 0, hdl_fm);    % STA 13
data(9) = fi(2323, 0, 12, 0, hdl_fm);    % LI 19
data(10) = fi(2574, 0, 12, 0, hdl_fm);    % STA 14
data(11) = fi(2555, 0, 12, 0, hdl_fm);    % LI 251
data(12) = fi(2575, 0, 12, 0, hdl_fm);    % STA 15
data(13) = fi(2319, 0, 12, 0, hdl_fm);    % LI 15
data(14) = fi(2576, 0, 12, 0, hdl_fm);    % STA 16
data(15) = fi(2558, 0, 12, 0, hdl_fm);    % LI 254
data(16) = fi(2577, 0, 12, 0, hdl_fm);    % STA 17
data(17) = fi(2306, 0, 12, 0, hdl_fm);    % LI 2
data(18) = fi(2578, 0, 12, 0, hdl_fm);    % STA 18
data(19) = fi(2315, 0, 12, 0, hdl_fm);    % LI 11
data(20) = fi(2579, 0, 12, 0, hdl_fm);    % STA 19
data(21) = fi(2324, 0, 12, 0, hdl_fm);    % LI 20
data(22) = fi(2580, 0, 12, 0, hdl_fm);    % STA 20
data(23) = fi(2314, 0, 12, 0, hdl_fm);    % LI 10
data(24) = fi(2581, 0, 12, 0, hdl_fm);    % STA 21
data(25) = fi(2305, 0, 12, 0, hdl_fm);    % LI 1
data(26) = fi(2562, 0, 12, 0, hdl_fm);    % STA 2
data(27) = fi(2305, 0, 12, 0, hdl_fm);    % LI 1
data(28) = fi(2563, 0, 12, 0, hdl_fm);    % STA 3
data(29) = fi(2305, 0, 12, 0, hdl_fm);    % LI 1
data(30) = fi(2564, 0, 12, 0, hdl_fm);    % STA 4
data(31) = fi(2, 0, 12, 0, hdl_fm);    % LDA 2
data(32) = fi(3704, 0, 12, 0, hdl_fm);    % CLC
data(33) = fi(1540, 0, 12, 0, hdl_fm);    % SUB 4
data(34) = fi(3704, 0, 12, 0, hdl_fm);    % CLC
data(35) = fi(1025, 0, 12, 0, hdl_fm);    % ADD 1
data(36) = fi(2565, 0, 12, 0, hdl_fm);    % STA 5
data(37) = fi(261, 0, 12, 0, hdl_fm);    % LDAI 5
data(38) = fi(2566, 0, 12, 0, hdl_fm);    % STA 6
data(39) = fi(2, 0, 12, 0, hdl_fm);    % LDA 2
data(40) = fi(3704, 0, 12, 0, hdl_fm);    % CLC
data(41) = fi(1025, 0, 12, 0, hdl_fm);    % ADD 1
data(42) = fi(2567, 0, 12, 0, hdl_fm);    % STA 7
data(43) = fi(263, 0, 12, 0, hdl_fm);    % LDAI 7
data(44) = fi(3704, 0, 12, 0, hdl_fm);    % CLC
data(45) = fi(1542, 0, 12, 0, hdl_fm);    % SUB 6
data(46) = fi(3330, 0, 12, 0, hdl_fm);    % BRA_N 2
data(47) = fi(2055, 0, 12, 0, hdl_fm);    % JMP 7
data(48) = fi(2304, 0, 12, 0, hdl_fm);    % LI 0
data(49) = fi(2563, 0, 12, 0, hdl_fm);    % STA 3
data(50) = fi(263, 0, 12, 0, hdl_fm);    % LDAI 7
data(51) = fi(2821, 0, 12, 0, hdl_fm);    % STAI 5
data(52) = fi(6, 0, 12, 0, hdl_fm);    % LDA 6
data(53) = fi(2823, 0, 12, 0, hdl_fm);    % STAI 7
data(54) = fi(2305, 0, 12, 0, hdl_fm);    % LI 1
data(55) = fi(3704, 0, 12, 0, hdl_fm);    % CLC
data(56) = fi(1026, 0, 12, 0, hdl_fm);    % ADD 2
data(57) = fi(2562, 0, 12, 0, hdl_fm);    % STA 2
data(58) = fi(0, 0, 12, 0, hdl_fm);    % LDA 0
data(59) = fi(3704, 0, 12, 0, hdl_fm);    % CLC
data(60) = fi(1538, 0, 12, 0, hdl_fm);    % SUB 2
data(61) = fi(3842, 0, 12, 0, hdl_fm);    % BRA_Z 2
data(62) = fi(2271, 0, 12, 0, hdl_fm);    % JMP -33
data(63) = fi(2305, 0, 12, 0, hdl_fm);    % LI 1
data(64) = fi(2564, 0, 12, 0, hdl_fm);    % STA 4
data(65) = fi(3, 0, 12, 0, hdl_fm);    % LDA 3
data(66) = fi(3704, 0, 12, 0, hdl_fm);    % CLC
data(67) = fi(1540, 0, 12, 0, hdl_fm);    % SUB 4
data(68) = fi(3842, 0, 12, 0, hdl_fm);    % BRA_Z 2
data(69) = fi(2260, 0, 12, 0, hdl_fm);    % JMP -44
data(70) = fi(2304, 0, 12, 0, hdl_fm);    % LI 0
data(71) = fi(2562, 0, 12, 0, hdl_fm);    % STA 2
data(72) = fi(257, 0, 12, 0, hdl_fm);    % LDAI 1
data(73) = fi(2815, 0, 12, 0, hdl_fm);    % STA 255
data(74) = fi(3696, 0, 12, 0, hdl_fm);    % PRINT
data(75) = fi(2305, 0, 12, 0, hdl_fm);    % LI 1
data(76) = fi(3704, 0, 12, 0, hdl_fm);    % CLC
data(77) = fi(1025, 0, 12, 0, hdl_fm);    % ADD 1
data(78) = fi(2561, 0, 12, 0, hdl_fm);    % STA 1
data(79) = fi(2305, 0, 12, 0, hdl_fm);    % LI 1
data(80) = fi(3704, 0, 12, 0, hdl_fm);    % CLC
data(81) = fi(1026, 0, 12, 0, hdl_fm);    % ADD 2
data(82) = fi(2562, 0, 12, 0, hdl_fm);    % STA 2
data(83) = fi(0, 0, 12, 0, hdl_fm);    % LDA 0
data(84) = fi(3704, 0, 12, 0, hdl_fm);    % CLC
data(85) = fi(1538, 0, 12, 0, hdl_fm);    % SUB 2
data(86) = fi(3842, 0, 12, 0, hdl_fm);    % BRA_Z 2
data(87) = fi(2289, 0, 12, 0, hdl_fm);    % JMP -15
data(88) = fi(3648, 0, 12, 0, hdl_fm);    % HLT


% Loading from memory
if(read == 1)
    instr_out = data(addr+1);
else
    instr_out = fi(0, 0, 12, 0, hdl_fm);
end

== matlab function hdlcodercpu_eml/CPU_Subsystem_8_bit/Instruction Register ==
  settings: updateMethod=DISCRETE  sampleTime=1
  settings: fimath=|
      | fimath(...
      | 'RoundMode', 'floor',...
      | 'OverflowMode', 'wrap',...
      | 'ProductMode', 'FullPrecision', 'ProductWordLength', 32,...
      | 'SumMode', 'FullPrecision', 'SumWordLength', 32,...
      | 'CastBeforeSum', true)
  data: func input fixdt(0,2,0); IR_out output; IR_in input fixdt(0,12,0)
function IR_out = Instruction_Reg(func, IR_in)
% A 12-bit Instruction Register with the following func:
% func == 0 => reset
% func == 1 => store into IR
% func == 2 => read from IR;
% otherwise, preserve old value and return 0

% HDL specific fimath
hdl_fm = fimath(...
'RoundMode', 'floor',...
'OverflowMode', 'wrap',...
'ProductMode', 'FullPrecision', 'ProductWordLength', 32,...
'SumMode', 'FullPrecision', 'SumWordLength', 32,...
'CastBeforeSum', true);


persistent IR_value;
if(isempty(IR_value))
    IR_value = fi(0, 0, 12, 0, hdl_fm);
end

IR_out = fi(0, 0, 12, 0, hdl_fm);
        
switch(uint8(func)) 
    case 0
        % reset
        IR_value = fi(0, 0, 12, 0, hdl_fm); 
    case 1
        % store into IR
        IR_value = IR_in;
    case 2
        % read IR
        IR_out = IR_value;
end

== matlab function hdlcodercpu_eml/CPU_Subsystem_8_bit/Program Counter ==
  settings: updateMethod=DISCRETE  sampleTime=1
  settings: fimath=|
      | fimath(...
      | 'RoundMode', 'floor',...
      | 'OverflowMode', 'wrap',...
      | 'ProductMode', 'FullPrecision', 'ProductWordLength', 32,...
      | 'SumMode', 'FullPrecision', 'SumWordLength', 32,...
      | 'CastBeforeSum', true)
  data: func input fixdt(0,2,0); addr_out output; addr_in input fixdt(0,8,0)
function addr_out = PC(func, addr_in)
% Program Counter
% func = 0 => reset PC
% func = 1 => load PC
% func = 2 => increment PC

% HDL specific fimath
hdl_fm = fimath(...
'RoundMode', 'floor',...
'OverflowMode', 'wrap',...
'ProductMode', 'FullPrecision', 'ProductWordLength', 32,...
'SumMode', 'FullPrecision', 'SumWordLength', 32,...
'CastBeforeSum', true);

persistent PC_value;
if(isempty(PC_value))
    PC_value = fi(0, 0, 8, 0, hdl_fm);
end

addr_out = fi(PC_value, 0, 8, 0, hdl_fm);

switch(uint8(func)) 
    case 0
        % reset
        PC_value = fi(0, 0, 8, 0, hdl_fm); 
    case 1
        % store into PC
        PC_value = addr_in;
    case 2
        % increment PC
        PC_value = fi(PC_value + 1, 0, 8, 0, hdl_fm);
end

== matlab function hdlcodercpu_eml/CPU_Subsystem_8_bit/Shifter (8-bit) ==
  settings: updateMethod=DISCRETE  sampleTime=1
  settings: fimath=|
      | fimath(...
      | 'RoundMode', 'floor',...
      | 'OverflowMode', 'wrap',...
      | 'ProductMode', 'FullPrecision', 'ProductWordLength', 32,...
      | 'SumMode', 'FullPrecision', 'SumWordLength', 32,...
      | 'CastBeforeSum', true)
  data: out_flags output; select input fixdt(0,2,0); shift_out output fixdt(1,8,0); input input fixdt(1,8,0); in_flags input
function [out_flags, shift_out] = Shifter(select, input, in_flags)
% An 8-bit shifter:
% select = 1 => shift left by 1 bit
% select = 2 => shift right by 1 bit
% otherwise, pass the input

% HDL specific fimath
hdl_fm = fimath(...
'RoundMode', 'floor',...
'OverflowMode', 'wrap',...
'ProductMode', 'FullPrecision', 'ProductWordLength', 32,...
'SumMode', 'FullPrecision', 'SumWordLength', 32,...
'CastBeforeSum', true);

% Overflow (V)
overflow = bitget(in_flags, 2);

% Carry (C)
c_out = bitget(in_flags, 4);

switch(uint8(select))
    case 1
        % shift left
        % affects C and V as well
        shift_out = bitsll(input, 1);
        % Carry (C)
        c_out = bitget(input, 8);
        % Overflow (V)
        overflow = bitxor(bitget(input, 8), bitget(input, 7));
    case 2
        % shift right
        shift_out = bitsra(input, 1);
    otherwise
        % pass the input
        shift_out = fi(input, 1, 8, 0, hdl_fm);
end

% Negativity  (N)
sign_bit = getmsb(shift_out); 

% Is Zero? (Z)
is_zero = uint8(~all(shift_out));
zero_ufix1 = fi(is_zero, 0, 1, 0, hdl_fm);

% Set [C, N, V, Z] in the flag register
out_flags = bitconcat(bitconcat(bitconcat(c_out, sign_bit), overflow), zero_ufix1);
